simulink model "simulator_model_controller_NE"  (R2023b)
settings: Solver=ode4  StartTime=0.0  StopTime=10  FixedStep=0.01  RelTol=1e-3
values from neighbouring files (symbols this model uses):
  f = 1/4    (= 0.25)    [main.m]
  Fv = 0.04    [main.m]
  g = Simulink.Parameter(9.81)    [main.m]
  I1 = Simulink.Parameter( (1/12)*m1.Value*(l1.Value^2) )    [main.m]
  I2 = Simulink.Parameter( (1/12)*m2.Value*(l2.Value^2) )    [main.m]
  Kd = sqrt(Kp/3)*3    [main.m]
  Kp = 10    [main.m]
  l1 = Simulink.Parameter(1)    [main.m]    (also in plot_robot.m = inputs(3); plot_robot_3links.m = inputs(4))
  l2 = Simulink.Parameter(1)    [main.m]    (also in plot_robot.m = inputs(4); plot_robot_3links.m = inputs(5))
  lc1 = Simulink.Parameter(l1.Value/2)    [main.m]
  lc2 = Simulink.Parameter(l2.Value/2)    [main.m]
  m1 = Simulink.Parameter(0.5)    [main.m]
  m2 = Simulink.Parameter(0.2)    [main.m]
  mx = 0.2    [main.m]
  my = 0.1    [main.m]
  px = 0.41    [main.m]
  py = 0.31    [main.m]
settings Model: Creator=Gabriel  LastModifiedBy=Bruno

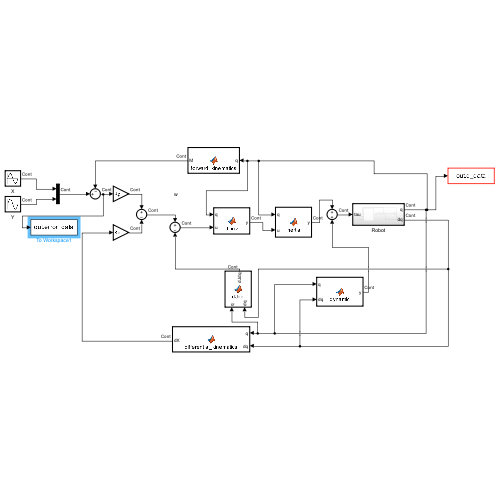
[thumbnail: Simulink's stored preview of the top-level diagram]
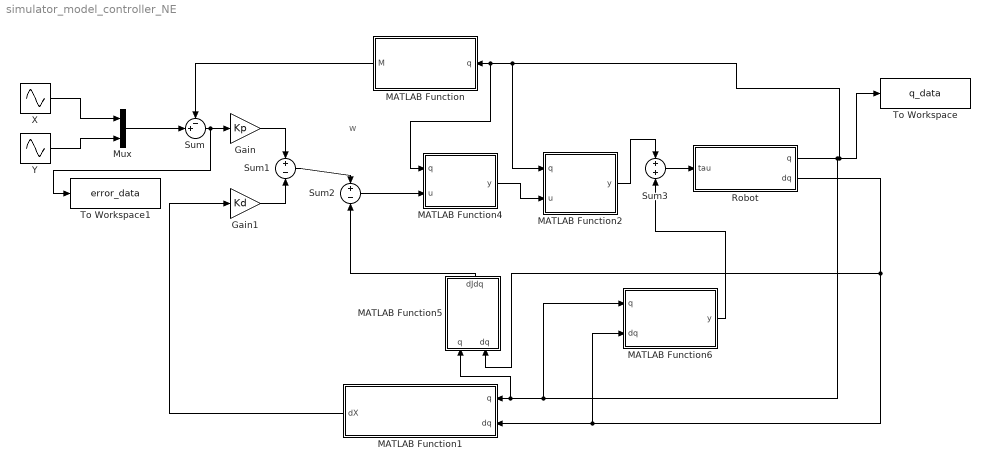
== system simulator_model_controller_NE ==
  note: w
  Gain : Gain  Gain=Kp
  Gain1 : Gain  Gain=Kd
  MATLAB Function : MATLAB Function  TreatAsAtomicUnit=on
  MATLAB Function1 : MATLAB Function  TreatAsAtomicUnit=on
  MATLAB Function2 : MATLAB Function  TreatAsAtomicUnit=on
  MATLAB Function4 : MATLAB Function  TreatAsAtomicUnit=on
  MATLAB Function5 : MATLAB Function  TreatAsAtomicUnit=on
  MATLAB Function6 : MATLAB Function  TreatAsAtomicUnit=on
  Mux : Mux  Inputs=2
  Robot : Subsystem
  Sum : Sum  Inputs=-+|
  Sum1 : Sum  Inputs=+-
  Sum2 : Sum  Inputs=+-
  Sum3 : Sum
  To Workspace : ToWorkspace  VariableName=q_data  SampleTime=-1
      settings: Save2DSignal=2-D array (concatenate along first dimension)
  To Workspace1 : ToWorkspace  VariableName=error_data  SampleTime=-1
      settings: Save2DSignal=2-D array (concatenate along first dimension)
  X : Sin  Amplitude=mx  Bias=px  Frequency=f*2*pi  Phase=pi/2  SampleTime=0
  Y : Sin  Amplitude=my  Bias=py  Frequency=f*pi*2  SampleTime=0
  wires:
  Robot/1(q) -> To Workspace/1, MATLAB Function2/1(q), MATLAB Function4/1(q), MATLAB Function/1(q), MATLAB Function6/1(q), MATLAB Function5/1(q), MATLAB Function1/1(q)
  MATLAB Function/1(M) -> Sum/1
  Gain1/1 -> Sum1/2
  Gain/1 -> Sum1/1
  Sum/1 -> To Workspace1/1, Gain/1
  Robot/2(dq) -> MATLAB Function5/2(dq), MATLAB Function6/2(dq), MATLAB Function1/2(dq)
  MATLAB Function1/1(dX) -> Gain1/1
  Sum1/1 -> Sum2/1
  MATLAB Function5/1(dJdq) -> Sum2/2
  Sum2/1 -> MATLAB Function4/2(u)
  MATLAB Function4/1(y) -> MATLAB Function2/2(u)
  MATLAB Function2/1(y) -> Sum3/1
  Sum3/1 -> Robot/1(tau)
  MATLAB Function6/1(y) -> Sum3/2
  X/1 -> Mux/1
  Y/1 -> Mux/2
  Mux/1 -> Sum/2

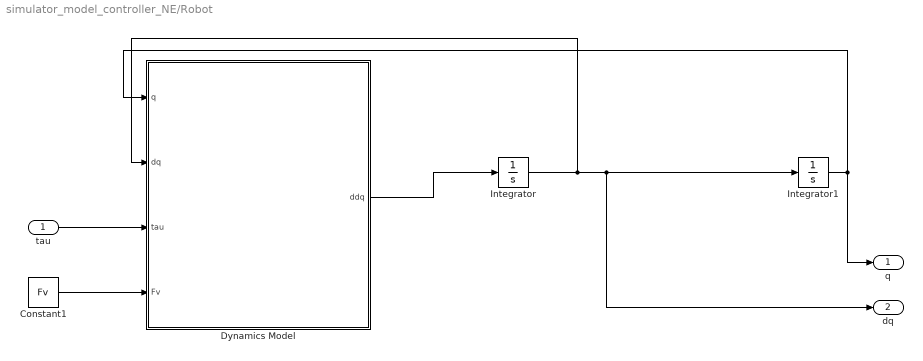
== system simulator_model_controller_NE/Robot ==
  tau : Inport
  Constant1 : Constant  Value=Fv
  Dynamics Model : MATLAB Function  TreatAsAtomicUnit=on
  Integrator : Integrator  InitialCondition=[0;0]
  Integrator1 : Integrator  InitialCondition=[pi/2;pi/4]
  q : Outport
  dq : Outport  Port=2
  wires:
  Integrator1/1 -> q/1, Dynamics Model/1(q)
  tau/1 -> Dynamics Model/3(tau)
  Dynamics Model/1(ddq) -> Integrator/1
  Integrator/1 -> Dynamics Model/2(dq), dq/1, Integrator1/1
  Constant1/1 -> Dynamics Model/4(Fv)

== matlab function simulator_model_controller_NE/Robot/Dynamics Model ==
  data: q input; ddq output; dq input; tau input; Fv input; m1 parameter; m2 parameter; l1 parameter; l2 parameter; lc1 parameter; lc2 parameter; I1 parameter; I2 parameter; g parameter
function ddq = dynamics(q,dq,tau,Fv, m1, m2, l1, l2, lc1, lc2, I1, I2, g)
M = mass_matrix(q(1),q(2),m1,m2,l1,l2,lc1,lc2,I1,I2);
C = coriolis_matrix(q(1),q(2),dq(1),dq(2),m1,m2,l1,l2,lc1,lc2);
G = gravity_vector(q(1),q(2),m1,m2,l1,l2,lc1,lc2,g);
J = Jacobian.linear_jacobian(q(1),q(2),l1,l2);

ddq = M \ (tau - C*dq - G - Fv * dq);

== matlab function simulator_model_controller_NE/MATLAB Function ==
  data: q input; l1 parameter; M output; l2 parameter
function M  = forward_kinematics(q, l1,l2)
    
    xt = l1*cos(q(1)) + l2*cos(q(1)+q(2)); 
    yt = l1*sin(q(1)) + l2*sin(q(1)+q(2));
    M = [xt; yt];

== matlab function simulator_model_controller_NE/MATLAB Function1 ==
  data: q input; dX output; dq input; l1 parameter; l2 parameter
function dX  = differential_kinematics(q,dq, l1, l2)
            q1=q(1);
            q2=q(2);
            dq1=dq(1);
            dq2=dq(2);
            dxt = -l1*sin(q1)*dq1 - l2*sin(q1+q2)*(dq1+dq2); 
            dyt = l1*cos(q1)*dq1 + l2*cos(q1+q2)*(dq1+dq2);
            dX = [dxt; dyt];

== matlab function simulator_model_controller_NE/MATLAB Function2 ==
  data: q input; u input; y output; m1 parameter; m2 parameter; l1 parameter; l2 parameter; lc1 parameter; lc2 parameter; I1 parameter; I2 parameter
function y = inertia(q,u, m1, m2, l1, l2, lc1, lc2, I1, I2)
M = mass_matrix(q(1),q(2),m1,m2,l1,l2,lc1,lc2,I1,I2);
y=M*u;

== matlab function simulator_model_controller_NE/MATLAB Function4 ==
  data: q input; u input; y output; l1 parameter; l2 parameter
function y = J_inv(q,u, l1, l2)
J=Jacobian.linear_jacobian(q(1),q(2),l1,l2);
J_inv = J \ eye(size(J));
y=J_inv*u;

== matlab function simulator_model_controller_NE/MATLAB Function5 ==
  data: q input; dJdq output; dq input; l1 parameter; l2 parameter
function dJdq = dJdq(q,dq, l1, l2)
dJ=Jacobian.differential_jacobian(q(1),q(2),dq(1),dq(2),l1,l2);
dJdq = dJ*dq;

== matlab function simulator_model_controller_NE/MATLAB Function6 ==
  data: q input; y output; dq input; m1 parameter; m2 parameter; l1 parameter; l2 parameter; lc1 parameter; lc2 parameter; g parameter
function y = dynamic(q,dq, m1, m2, l1, l2, lc1, lc2, g)
C = coriolis_matrix(q(1),q(2),dq(1),dq(2),m1,m2,l1,l2,lc1,lc2);
V = C*dq;
G = gravity_vector(q(1),q(2),m1,m2,l1,l2,lc1,lc2,g);
y=V+G;
